simulink model "s_c_nbe_m32k"  (R2018a)
settings: Solver=VariableStepDiscrete  StartTime=0.0  StopTime=1000  RelTol=1e-3
undefined symbols (not defined in the file): fft_stages, n_taps, output_bits, pfb_coeff_gen_calc, xengbits
libraries: xbsIndex_r4 x23714, casper_library_misc x17, xps_library x4, casper_library_scopes x4, xbsReplacements_r4 x4
(part 125 of 171)

== system s_c_nbe_m32k/nb_pfb/pfb_fir_generic2/pfb_fir_taps/tap_delays ==
  addra : Inport
  dina : Inport  Port=2
  wea : Inport  Port=3
  addrb : Inport  Port=4
  dinb : Inport  Port=5
  web : Inport  Port=6
  A_bussify0 : Subsystem  mask(bus_create){inputNum=108}
      mask prompts: inputNum "Number of inputs:"
      mask init:
      | bus_create_init(gcb,...
      |     'inputNum', inputNum);
  B_bussify0 : Subsystem  mask(bus_create){inputNum=108}
      mask prompts: inputNum "Number of inputs:"
      mask init:
      | bus_create_init(gcb,...
      |     'inputNum', inputNum);
  alsbs_slice : xbsIndex_r4/Slice  nbits=15  boolean_output=off  mode=Lower Bit Location + Width  bit1=0  base1=LSB of Input  bit0=0  base0=LSB of Input  dbl_ovrd=off  block_type=slice
  blsbs_slice : xbsIndex_r4/Slice  nbits=15  boolean_output=off  mode=Lower Bit Location + Width  bit1=0  base1=LSB of Input  bit0=0  base0=LSB of Input  dbl_ovrd=off  block_type=slice
  bram0_{0..107} (108 alike) : xbsIndex_r4/Dual Port RAM  depth=32768  initVector=getfield(get_param(gcb, 'UserData'), 'initVector')  distributed_mem=Block RAM  init_a=0  init_b=0  rst_a=off  rst_b=off  en_a=off  en_b=off  latency=7  write_mode_A=Read Before Write  write_mode_B=Read Before Write  optimize=Speed  dbl_ovrd=off  block_type=dpram
  ddina0 : xbsIndex_r4/Delay  rst=off  infoeditControl=Selection of Reset will increase slice count due to use of real FFs and instead of SRLs  en=off  latency=0  reg_retiming=on  dbl_ovrd=off  block_type=delay
  ddinb0 : xbsIndex_r4/Delay  rst=off  infoeditControl=Selection of Reset will increase slice count due to use of real FFs and instead of SRLs  en=off  latency=4  reg_retiming=off  dbl_ovrd=off  block_type=delay
  debus_addra0 : Subsystem  mask(bus_expand){mode=divisions of equal size, outputNum=108, outputWidth=[15 15 15 15 15 15 15 15 15 15 15 15 15 15 15 15 15 15 15 15 15 15 15 15 15 15 15 15 15 15 15 15 15 15 15 15 15 15 15 15 15 15 15 15 15 15 15 15 15 15 15 15 15 15 15 15 15 15 15 15 15 15 15 15 15 15 15 15 15 15 15 15 15 15 15 15 15 15 15 15 15 15 15 15 15 15 15 15 15 15 15 15 15 15 15 15 15 15 15 15 15 15 15 15 15 15 15 15], outputBinaryPt=[0 0 0 0 0 0 0 0 0 0 0 0 0 0 0 0 0 0 0 0 0 0 0 0 0 0 0 0 0 0 0 0 0 0 0 0 0 0 0 0 0 0 0 0 0 0 0 0 0 0 0 0 0 0 0 0 0 0 0 0 0 0 0 0 0 0 0 0 0 0 0 0 0 0 0 0 0 0 0 0 0 0 0 0 0 0 0 0 0 0 0 0 0 0 0 0 0 0 0 0 0 0 0 0 0 0 0 0], outputArithmeticType=[0 0 0 0 0 0 0 0 0 0 0 0 0 0 0 0 0 0 0 0 0 0 0 0 0 0 0 0 0 0 0 0 0 0 0 0 0 0 0 0 0 0 0 0 0 0 0 0 0 0 0 0 0 0 0 0 0 0 0 0 0 0 0 0 0 0 0 0 0 0 0 0 0 0 0 0 0 0 0 0 0 0 0 0 0 0 0 0 0 0 0 0 0 0 0 0 0 0 0 0 0 0 0 0 0 0 0 0], show_format=on, outputToWorkspace=off, variablePrefix=, outputToModelAsWell=on}
      mask prompts: outputNum "Number of outputs:"; outputWidth "Output width:"; outputBinaryPt "Output binary point position:"; outputArithmeticType "Output arithmetic type (ufix=0, fix=1, bool=2):"; show_format "Print format string?"; outputToWorkspace "Output to workspace?"; variablePrefix "Variable name prefix:"; outputToModelAsWell "Output to model as well?"
      mask help:
      | Expands a 'bus' made using a bus_create or Xilinx
      | concat block.
      | The input will be divided into the specified number
      | of outputs with the specified arithmetic types.
      | Divisions are made from most significant bit.
      mask init: same as s_c_nbe_m32k/bus_expand1
      settings: AttributesFormatString=108 outputs: uf15.0,uf15.0,uf15.0,uf15.0,uf15.0,uf15.0,uf15.0,uf15.0,uf15.0,uf15.0,uf15.0,uf15.0,uf15.0,uf15.0,uf15.0,uf15.0,uf15.0,uf15.0,uf15.0,uf15.0,uf15.0,uf15.0,uf15.0,uf15.0,uf15.0,uf15.0,uf15.0,uf15.0,uf15.0,uf15.0,uf15.0,uf15.0,uf15.0,uf15.0,uf15.0,uf15.0,uf15.0,uf15.0,uf15.0,uf15.0,uf15.0,uf15.0,uf15.0,uf15.0,uf15.0,uf15.0,uf15.0,uf15.0,uf15.0,uf15.0,uf15.0,uf15.0,uf15.0,uf15.0,uf15.0,uf15.0,uf15.0,uf15.0,uf15.0,uf15.0,uf15.0,uf15.0,uf15.0,uf15.0,uf15.0,uf15.0,uf15.0,uf15.0,uf15.0,uf15.0,uf15.0,uf15.0,uf15.0,uf15.0,uf15.0,uf15.0,uf15.0,uf15.0,uf15.0,uf15.0,uf15.0,uf15.0,uf15.0,uf15.0,uf15.0,uf15.0,uf15.0,uf15.0,uf15.0,uf15.0,uf15.0,uf15.0,uf15.0,uf15.0,uf15.0,uf15.0,uf15.0,uf15.0,uf15.0,uf15.0,uf15.0,uf15.0,uf15.0,uf15.0,uf15.0,uf15.0,uf15.0,uf15.0,
      mask TypeOptions mode: divisions of equal size | divisions of arbitrary size
      mask Callback mode: bus_expand_callback();
      mask Callback outputWidth: bus_expand_callback();
      mask Callback outputToWorkspace: bus_expand_callback();
  debus_addrb0 : Subsystem  mask(bus_expand){mode=divisions of equal size, outputNum=108, outputWidth=[15 15 15 15 15 15 15 15 15 15 15 15 15 15 15 15 15 15 15 15 15 15 15 15 15 15 15 15 15 15 15 15 15 15 15 15 15 15 15 15 15 15 15 15 15 15 15 15 15 15 15 15 15 15 15 15 15 15 15 15 15 15 15 15 15 15 15 15 15 15 15 15 15 15 15 15 15 15 15 15 15 15 15 15 15 15 15 15 15 15 15 15 15 15 15 15 15 15 15 15 15 15 15 15 15 15 15 15], outputBinaryPt=[0 0 0 0 0 0 0 0 0 0 0 0 0 0 0 0 0 0 0 0 0 0 0 0 0 0 0 0 0 0 0 0 0 0 0 0 0 0 0 0 0 0 0 0 0 0 0 0 0 0 0 0 0 0 0 0 0 0 0 0 0 0 0 0 0 0 0 0 0 0 0 0 0 0 0 0 0 0 0 0 0 0 0 0 0 0 0 0 0 0 0 0 0 0 0 0 0 0 0 0 0 0 0 0 0 0 0 0], outputArithmeticType=[0 0 0 0 0 0 0 0 0 0 0 0 0 0 0 0 0 0 0 0 0 0 0 0 0 0 0 0 0 0 0 0 0 0 0 0 0 0 0 0 0 0 0 0 0 0 0 0 0 0 0 0 0 0 0 0 0 0 0 0 0 0 0 0 0 0 0 0 0 0 0 0 0 0 0 0 0 0 0 0 0 0 0 0 0 0 0 0 0 0 0 0 0 0 0 0 0 0 0 0 0 0 0 0 0 0 0 0], show_format=on, outputToWorkspace=off, variablePrefix=, outputToModelAsWell=on}
      mask prompts: outputNum "Number of outputs:"; outputWidth "Output width:"; outputBinaryPt "Output binary point position:"; outputArithmeticType "Output arithmetic type (ufix=0, fix=1, bool=2):"; show_format "Print format string?"; outputToWorkspace "Output to workspace?"; variablePrefix "Variable name prefix:"; outputToModelAsWell "Output to model as well?"
      mask help:
      | Expands a 'bus' made using a bus_create or Xilinx
      | concat block.
      | The input will be divided into the specified number
      | of outputs with the specified arithmetic types.
      | Divisions are made from most significant bit.
      mask init: same as s_c_nbe_m32k/bus_expand1
      settings: AttributesFormatString=108 outputs: uf15.0,uf15.0,uf15.0,uf15.0,uf15.0,uf15.0,uf15.0,uf15.0,uf15.0,uf15.0,uf15.0,uf15.0,uf15.0,uf15.0,uf15.0,uf15.0,uf15.0,uf15.0,uf15.0,uf15.0,uf15.0,uf15.0,uf15.0,uf15.0,uf15.0,uf15.0,uf15.0,uf15.0,uf15.0,uf15.0,uf15.0,uf15.0,uf15.0,uf15.0,uf15.0,uf15.0,uf15.0,uf15.0,uf15.0,uf15.0,uf15.0,uf15.0,uf15.0,uf15.0,uf15.0,uf15.0,uf15.0,uf15.0,uf15.0,uf15.0,uf15.0,uf15.0,uf15.0,uf15.0,uf15.0,uf15.0,uf15.0,uf15.0,uf15.0,uf15.0,uf15.0,uf15.0,uf15.0,uf15.0,uf15.0,uf15.0,uf15.0,uf15.0,uf15.0,uf15.0,uf15.0,uf15.0,uf15.0,uf15.0,uf15.0,uf15.0,uf15.0,uf15.0,uf15.0,uf15.0,uf15.0,uf15.0,uf15.0,uf15.0,uf15.0,uf15.0,uf15.0,uf15.0,uf15.0,uf15.0,uf15.0,uf15.0,uf15.0,uf15.0,uf15.0,uf15.0,uf15.0,uf15.0,uf15.0,uf15.0,uf15.0,uf15.0,uf15.0,uf15.0,uf15.0,uf15.0,uf15.0,uf15.0,
      mask TypeOptions mode: divisions of equal size | divisions of arbitrary size
      mask Callback mode: bus_expand_callback();
      mask Callback outputWidth: bus_expand_callback();
      mask Callback outputToWorkspace: bus_expand_callback();
  debus_dina0 : Subsystem  mask(bus_expand){mode=divisions of arbitrary size, outputNum=1, outputWidth=[1 1 1 1 1 1 1 1 1 1 1 1 1 1 1 1 1 1 1 1 1 1 1 1 1 1 1 1 1 1 1 1 1 1 1 1 1 1 1 1 1 1 1 1 1 1 1 1 1 1 1 1 1 1 1 1 1 1 1 1 1 1 1 1 1 1 1 1 1 1 1 1 1 1 1 1 1 1 1 1 1 1 1 1 1 1 1 1 1 1 1 1 1 1 1 1 1 1 1 1 1 1 1 1 1 1 1 1], outputBinaryPt=[0 0 0 0 0 0 0 0 0 0 0 0 0 0 0 0 0 0 0 0 0 0 0 0 0 0 0 0 0 0 0 0 0 0 0 0 0 0 0 0 0 0 0 0 0 0 0 0 0 0 0 0 0 0 0 0 0 0 0 0 0 0 0 0 0 0 0 0 0 0 0 0 0 0 0 0 0 0 0 0 0 0 0 0 0 0 0 0 0 0 0 0 0 0 0 0 0 0 0 0 0 0 0 0 0 0 0 0], outputArithmeticType=[0 0 0 0 0 0 0 0 0 0 0 0 0 0 0 0 0 0 0 0 0 0 0 0 0 0 0 0 0 0 0 0 0 0 0 0 0 0 0 0 0 0 0 0 0 0 0 0 0 0 0 0 0 0 0 0 0 0 0 0 0 0 0 0 0 0 0 0 0 0 0 0 0 0 0 0 0 0 0 0 0 0 0 0 0 0 0 0 0 0 0 0 0 0 0 0 0 0 0 0 0 0 0 0 0 0 0 0], show_format=on, outputToWorkspace=off, variablePrefix=, outputToModelAsWell=on}
      mask prompts: outputNum "Number of outputs:"; outputWidth "Output width [msb ... lsb]:"; outputBinaryPt "Output binary point position [msb ... lsb]:"; outputArithmeticType "Output arithmetic type (ufix=0, fix=1, bool=2) [msb ... lsb]:"; show_format "Print format string?"; outputToWorkspace "Output to workspace?"; variablePrefix "Variable name prefix:"; outputToModelAsWell "Output to model as well?"
      mask help:
      | Expands a 'bus' made using a bus_create or Xilinx
      | concat block.
      | The input will be divided into the specified number
      | of outputs with the specified arithmetic types.
      | Divisions are made from most significant bit.
      mask init: same as s_c_nbe_m32k/bus_expand1
      settings: AttributesFormatString=108 outputs: uf1.0,uf1.0,uf1.0,uf1.0,uf1.0,uf1.0,uf1.0,uf1.0,uf1.0,uf1.0,uf1.0,uf1.0,uf1.0,uf1.0,uf1.0,uf1.0,uf1.0,uf1.0,uf1.0,uf1.0,uf1.0,uf1.0,uf1.0,uf1.0,uf1.0,uf1.0,uf1.0,uf1.0,uf1.0,uf1.0,uf1.0,uf1.0,uf1.0,uf1.0,uf1.0,uf1.0,uf1.0,uf1.0,uf1.0,uf1.0,uf1.0,uf1.0,uf1.0,uf1.0,uf1.0,uf1.0,uf1.0,uf1.0,uf1.0,uf1.0,uf1.0,uf1.0,uf1.0,uf1.0,uf1.0,uf1.0,uf1.0,uf1.0,uf1.0,uf1.0,uf1.0,uf1.0,uf1.0,uf1.0,uf1.0,uf1.0,uf1.0,uf1.0,uf1.0,uf1.0,uf1.0,uf1.0,uf1.0,uf1.0,uf1.0,uf1.0,uf1.0,uf1.0,uf1.0,uf1.0,uf1.0,uf1.0,uf1.0,uf1.0,uf1.0,uf1.0,uf1.0,uf1.0,uf1.0,uf1.0,uf1.0,uf1.0,uf1.0,uf1.0,uf1.0,uf1.0,uf1.0,uf1.0,uf1.0,uf1.0,uf1.0,uf1.0,uf1.0,uf1.0,uf1.0,uf1.0,uf1.0,uf1.0,
      mask TypeOptions mode: divisions of equal size | divisions of arbitrary size
      mask Callback mode: bus_expand_callback();
      mask Callback outputWidth: bus_expand_callback();
      mask Callback outputToWorkspace: bus_expand_callback();
  debus_dinb0 : Subsystem  mask(bus_expand){mode=divisions of arbitrary size, outputNum=1, outputWidth=[1 1 1 1 1 1 1 1 1 1 1 1 1 1 1 1 1 1 1 1 1 1 1 1 1 1 1 1 1 1 1 1 1 1 1 1 1 1 1 1 1 1 1 1 1 1 1 1 1 1 1 1 1 1 1 1 1 1 1 1 1 1 1 1 1 1 1 1 1 1 1 1 1 1 1 1 1 1 1 1 1 1 1 1 1 1 1 1 1 1 1 1 1 1 1 1 1 1 1 1 1 1 1 1 1 1 1 1], outputBinaryPt=[0 0 0 0 0 0 0 0 0 0 0 0 0 0 0 0 0 0 0 0 0 0 0 0 0 0 0 0 0 0 0 0 0 0 0 0 0 0 0 0 0 0 0 0 0 0 0 0 0 0 0 0 0 0 0 0 0 0 0 0 0 0 0 0 0 0 0 0 0 0 0 0 0 0 0 0 0 0 0 0 0 0 0 0 0 0 0 0 0 0 0 0 0 0 0 0 0 0 0 0 0 0 0 0 0 0 0 0], outputArithmeticType=[0 0 0 0 0 0 0 0 0 0 0 0 0 0 0 0 0 0 0 0 0 0 0 0 0 0 0 0 0 0 0 0 0 0 0 0 0 0 0 0 0 0 0 0 0 0 0 0 0 0 0 0 0 0 0 0 0 0 0 0 0 0 0 0 0 0 0 0 0 0 0 0 0 0 0 0 0 0 0 0 0 0 0 0 0 0 0 0 0 0 0 0 0 0 0 0 0 0 0 0 0 0 0 0 0 0 0 0], show_format=on, outputToWorkspace=off, variablePrefix=, outputToModelAsWell=on}
      mask prompts: outputNum "Number of outputs:"; outputWidth "Output width [msb ... lsb]:"; outputBinaryPt "Output binary point position [msb ... lsb]:"; outputArithmeticType "Output arithmetic type (ufix=0, fix=1, bool=2) [msb ... lsb]:"; show_format "Print format string?"; outputToWorkspace "Output to workspace?"; variablePrefix "Variable name prefix:"; outputToModelAsWell "Output to model as well?"
      mask help:
      | Expands a 'bus' made using a bus_create or Xilinx
      | concat block.
      | The input will be divided into the specified number
      | of outputs with the specified arithmetic types.
      | Divisions are made from most significant bit.
      mask init: same as s_c_nbe_m32k/bus_expand1
      settings: AttributesFormatString=108 outputs: uf1.0,uf1.0,uf1.0,uf1.0,uf1.0,uf1.0,uf1.0,uf1.0,uf1.0,uf1.0,uf1.0,uf1.0,uf1.0,uf1.0,uf1.0,uf1.0,uf1.0,uf1.0,uf1.0,uf1.0,uf1.0,uf1.0,uf1.0,uf1.0,uf1.0,uf1.0,uf1.0,uf1.0,uf1.0,uf1.0,uf1.0,uf1.0,uf1.0,uf1.0,uf1.0,uf1.0,uf1.0,uf1.0,uf1.0,uf1.0,uf1.0,uf1.0,uf1.0,uf1.0,uf1.0,uf1.0,uf1.0,uf1.0,uf1.0,uf1.0,uf1.0,uf1.0,uf1.0,uf1.0,uf1.0,uf1.0,uf1.0,uf1.0,uf1.0,uf1.0,uf1.0,uf1.0,uf1.0,uf1.0,uf1.0,uf1.0,uf1.0,uf1.0,uf1.0,uf1.0,uf1.0,uf1.0,uf1.0,uf1.0,uf1.0,uf1.0,uf1.0,uf1.0,uf1.0,uf1.0,uf1.0,uf1.0,uf1.0,uf1.0,uf1.0,uf1.0,uf1.0,uf1.0,uf1.0,uf1.0,uf1.0,uf1.0,uf1.0,uf1.0,uf1.0,uf1.0,uf1.0,uf1.0,uf1.0,uf1.0,uf1.0,uf1.0,uf1.0,uf1.0,uf1.0,uf1.0,uf1.0,uf1.0,
      mask TypeOptions mode: divisions of equal size | divisions of arbitrary size
      mask Callback mode: bus_expand_callback();
      mask Callback outputWidth: bus_expand_callback();
      mask Callback outputToWorkspace: bus_expand_callback();
  debus_wea0 : Subsystem  mask(bus_expand){mode=divisions of equal size, outputNum=108, outputWidth=[1 1 1 1 1 1 1 1 1 1 1 1 1 1 1 1 1 1 1 1 1 1 1 1 1 1 1 1 1 1 1 1 1 1 1 1 1 1 1 1 1 1 1 1 1 1 1 1 1 1 1 1 1 1 1 1 1 1 1 1 1 1 1 1 1 1 1 1 1 1 1 1 1 1 1 1 1 1 1 1 1 1 1 1 1 1 1 1 1 1 1 1 1 1 1 1 1 1 1 1 1 1 1 1 1 1 1 1], outputBinaryPt=[0 0 0 0 0 0 0 0 0 0 0 0 0 0 0 0 0 0 0 0 0 0 0 0 0 0 0 0 0 0 0 0 0 0 0 0 0 0 0 0 0 0 0 0 0 0 0 0 0 0 0 0 0 0 0 0 0 0 0 0 0 0 0 0 0 0 0 0 0 0 0 0 0 0 0 0 0 0 0 0 0 0 0 0 0 0 0 0 0 0 0 0 0 0 0 0 0 0 0 0 0 0 0 0 0 0 0 0], outputArithmeticType=[2 2 2 2 2 2 2 2 2 2 2 2 2 2 2 2 2 2 2 2 2 2 2 2 2 2 2 2 2 2 2 2 2 2 2 2 2 2 2 2 2 2 2 2 2 2 2 2 2 2 2 2 2 2 2 2 2 2 2 2 2 2 2 2 2 2 2 2 2 2 2 2 2 2 2 2 2 2 2 2 2 2 2 2 2 2 2 2 2 2 2 2 2 2 2 2 2 2 2 2 2 2 2 2 2 2 2 2], show_format=on, outputToWorkspace=off, variablePrefix=, outputToModelAsWell=on}
      mask prompts: outputNum "Number of outputs:"; outputWidth "Output width:"; outputBinaryPt "Output binary point position:"; outputArithmeticType "Output arithmetic type (ufix=0, fix=1, bool=2):"; show_format "Print format string?"; outputToWorkspace "Output to workspace?"; variablePrefix "Variable name prefix:"; outputToModelAsWell "Output to model as well?"
      mask help:
      | Expands a 'bus' made using a bus_create or Xilinx
      | concat block.
      | The input will be divided into the specified number
      | of outputs with the specified arithmetic types.
      | Divisions are made from most significant bit.
      mask init: same as s_c_nbe_m32k/bus_expand1
      settings: AttributesFormatString=108 outputs: b,b,b,b,b,b,b,b,b,b,b,b,b,b,b,b,b,b,b,b,b,b,b,b,b,b,b,b,b,b,b,b,b,b,b,b,b,b,b,b,b,b,b,b,b,b,b,b,b,b,b,b,b,b,b,b,b,b,b,b,b,b,b,b,b,b,b,b,b,b,b,b,b,b,b,b,b,b,b,b,b,b,b,b,b,b,b,b,b,b,b,b,b,b,b,b,b,b,b,b,b,b,b,b,b,b,b,b,
      mask TypeOptions mode: divisions of equal size | divisions of arbitrary size
      mask Callback mode: bus_expand_callback();
      mask Callback outputWidth: bus_expand_callback();
      mask Callback outputToWorkspace: bus_expand_callback();
  debus_web0 : Subsystem  mask(bus_expand){mode=divisions of equal size, outputNum=108, outputWidth=[1 1 1 1 1 1 1 1 1 1 1 1 1 1 1 1 1 1 1 1 1 1 1 1 1 1 1 1 1 1 1 1 1 1 1 1 1 1 1 1 1 1 1 1 1 1 1 1 1 1 1 1 1 1 1 1 1 1 1 1 1 1 1 1 1 1 1 1 1 1 1 1 1 1 1 1 1 1 1 1 1 1 1 1 1 1 1 1 1 1 1 1 1 1 1 1 1 1 1 1 1 1 1 1 1 1 1 1], outputBinaryPt=[0 0 0 0 0 0 0 0 0 0 0 0 0 0 0 0 0 0 0 0 0 0 0 0 0 0 0 0 0 0 0 0 0 0 0 0 0 0 0 0 0 0 0 0 0 0 0 0 0 0 0 0 0 0 0 0 0 0 0 0 0 0 0 0 0 0 0 0 0 0 0 0 0 0 0 0 0 0 0 0 0 0 0 0 0 0 0 0 0 0 0 0 0 0 0 0 0 0 0 0 0 0 0 0 0 0 0 0], outputArithmeticType=[2 2 2 2 2 2 2 2 2 2 2 2 2 2 2 2 2 2 2 2 2 2 2 2 2 2 2 2 2 2 2 2 2 2 2 2 2 2 2 2 2 2 2 2 2 2 2 2 2 2 2 2 2 2 2 2 2 2 2 2 2 2 2 2 2 2 2 2 2 2 2 2 2 2 2 2 2 2 2 2 2 2 2 2 2 2 2 2 2 2 2 2 2 2 2 2 2 2 2 2 2 2 2 2 2 2 2 2], show_format=on, outputToWorkspace=off, variablePrefix=, outputToModelAsWell=on}
      mask prompts: outputNum "Number of outputs:"; outputWidth "Output width:"; outputBinaryPt "Output binary point position:"; outputArithmeticType "Output arithmetic type (ufix=0, fix=1, bool=2):"; show_format "Print format string?"; outputToWorkspace "Output to workspace?"; variablePrefix "Variable name prefix:"; outputToModelAsWell "Output to model as well?"
      mask help:
      | Expands a 'bus' made using a bus_create or Xilinx
      | concat block.
      | The input will be divided into the specified number
      | of outputs with the specified arithmetic types.
      | Divisions are made from most significant bit.
      mask init: same as s_c_nbe_m32k/bus_expand1
      settings: AttributesFormatString=108 outputs: b,b,b,b,b,b,b,b,b,b,b,b,b,b,b,b,b,b,b,b,b,b,b,b,b,b,b,b,b,b,b,b,b,b,b,b,b,b,b,b,b,b,b,b,b,b,b,b,b,b,b,b,b,b,b,b,b,b,b,b,b,b,b,b,b,b,b,b,b,b,b,b,b,b,b,b,b,b,b,b,b,b,b,b,b,b,b,b,b,b,b,b,b,b,b,b,b,b,b,b,b,b,b,b,b,b,b,b,
      mask TypeOptions mode: divisions of equal size | divisions of arbitrary size
      mask Callback mode: bus_expand_callback();
      mask Callback outputWidth: bus_expand_callback();
      mask Callback outputToWorkspace: bus_expand_callback();
  rep_addra0 : Subsystem  mask(bus_replicate){replication=108, csp_latency=4, misc=off, implementation=core}
      mask prompts: replication "replication factor"; csp_latency "latency"; misc "misc support"; implementation "delay implementation"
      mask help: Output bus formed by replicating input bus a number of times
      mask init:
      | bus_replicate_init(gcb, ...
      |     'replication', replication, ...
      |     'csp_latency', csp_latency, ...
      |     'implementation', implementation, ...
      |     'misc', misc);
      mask TypeOptions implementation: core | behavioral
  rep_addrb0 : Subsystem  mask(bus_replicate){replication=108, csp_latency=4, misc=off, implementation=core}
      mask prompts: replication "replication factor"; csp_latency "latency"; misc "misc support"; implementation "delay implementation"
      mask help: Output bus formed by replicating input bus a number of times
      mask init:
      | bus_replicate_init(gcb, ...
      |     'replication', replication, ...
      |     'csp_latency', csp_latency, ...
      |     'implementation', implementation, ...
      |     'misc', misc);
      mask TypeOptions implementation: core | behavioral
  rep_wea0 : Subsystem  mask(bus_replicate){replication=108, csp_latency=0, misc=off, implementation=behavioral}
      mask prompts: replication "replication factor"; csp_latency "latency"; misc "misc support"; implementation "delay implementation"
      mask help: Output bus formed by replicating input bus a number of times
      mask init:
      | bus_replicate_init(gcb, ...
      |     'replication', replication, ...
      |     'csp_latency', csp_latency, ...
      |     'implementation', implementation, ...
      |     'misc', misc);
      mask TypeOptions implementation: core | behavioral
  rep_web0 : Subsystem  mask(bus_replicate){replication=108, csp_latency=4, misc=off, implementation=core}
      mask prompts: replication "replication factor"; csp_latency "latency"; misc "misc support"; implementation "delay implementation"
      mask help: Output bus formed by replicating input bus a number of times
      mask init:
      | bus_replicate_init(gcb, ...
      |     'replication', replication, ...
      |     'csp_latency', csp_latency, ...
      |     'implementation', implementation, ...
      |     'misc', misc);
      mask TypeOptions implementation: core | behavioral
  A : Outport
  B : Outport  Port=2
  wires:
  B_bussify0/1(bus_out) -> B/1
  A_bussify0/1(bus_out) -> A/1
  bram0_107/2 -> B_bussify0/108(in108)
  bram0_107/1 -> A_bussify0/108(in108)
  bram0_106/2 -> B_bussify0/107(in107)
  bram0_106/1 -> A_bussify0/107(in107)
  bram0_105/2 -> B_bussify0/106(in106)
  bram0_105/1 -> A_bussify0/106(in106)
  bram0_104/2 -> B_bussify0/105(in105)
  bram0_104/1 -> A_bussify0/105(in105)
  bram0_103/2 -> B_bussify0/104(in104)
  bram0_103/1 -> A_bussify0/104(in104)
  bram0_102/2 -> B_bussify0/103(in103)
  bram0_102/1 -> A_bussify0/103(in103)
  bram0_101/2 -> B_bussify0/102(in102)
  bram0_101/1 -> A_bussify0/102(in102)
  bram0_100/2 -> B_bussify0/101(in101)
  bram0_100/1 -> A_bussify0/101(in101)
  bram0_99/2 -> B_bussify0/100(in100)
  bram0_99/1 -> A_bussify0/100(in100)
  bram0_98/2 -> B_bussify0/99(in99)
  bram0_98/1 -> A_bussify0/99(in99)
  bram0_97/2 -> B_bussify0/98(in98)
  bram0_97/1 -> A_bussify0/98(in98)
  bram0_96/2 -> B_bussify0/97(in97)
  bram0_96/1 -> A_bussify0/97(in97)
  bram0_95/2 -> B_bussify0/96(in96)
  bram0_95/1 -> A_bussify0/96(in96)
  bram0_94/2 -> B_bussify0/95(in95)
  bram0_94/1 -> A_bussify0/95(in95)
  bram0_93/2 -> B_bussify0/94(in94)
  bram0_93/1 -> A_bussify0/94(in94)
  bram0_92/2 -> B_bussify0/93(in93)
  bram0_92/1 -> A_bussify0/93(in93)
  bram0_91/2 -> B_bussify0/92(in92)
  bram0_91/1 -> A_bussify0/92(in92)
  bram0_90/2 -> B_bussify0/91(in91)
  bram0_90/1 -> A_bussify0/91(in91)
  bram0_89/2 -> B_bussify0/90(in90)
  bram0_89/1 -> A_bussify0/90(in90)
  bram0_88/2 -> B_bussify0/89(in89)
  bram0_88/1 -> A_bussify0/89(in89)
  bram0_87/2 -> B_bussify0/88(in88)
  bram0_87/1 -> A_bussify0/88(in88)
  bram0_86/2 -> B_bussify0/87(in87)
  bram0_86/1 -> A_bussify0/87(in87)
  bram0_85/2 -> B_bussify0/86(in86)
  bram0_85/1 -> A_bussify0/86(in86)
  bram0_84/2 -> B_bussify0/85(in85)
  bram0_84/1 -> A_bussify0/85(in85)
  bram0_83/2 -> B_bussify0/84(in84)
  bram0_83/1 -> A_bussify0/84(in84)
  bram0_82/2 -> B_bussify0/83(in83)
  bram0_82/1 -> A_bussify0/83(in83)
  bram0_81/2 -> B_bussify0/82(in82)
  bram0_81/1 -> A_bussify0/82(in82)
  bram0_80/2 -> B_bussify0/81(in81)
  bram0_80/1 -> A_bussify0/81(in81)
  bram0_79/2 -> B_bussify0/80(in80)
  bram0_79/1 -> A_bussify0/80(in80)
  bram0_78/2 -> B_bussify0/79(in79)
  bram0_78/1 -> A_bussify0/79(in79)
  bram0_77/2 -> B_bussify0/78(in78)
  bram0_77/1 -> A_bussify0/78(in78)
  bram0_76/2 -> B_bussify0/77(in77)
  bram0_76/1 -> A_bussify0/77(in77)
  bram0_75/2 -> B_bussify0/76(in76)
  bram0_75/1 -> A_bussify0/76(in76)
  bram0_74/2 -> B_bussify0/75(in75)
  bram0_74/1 -> A_bussify0/75(in75)
  bram0_73/2 -> B_bussify0/74(in74)
  bram0_73/1 -> A_bussify0/74(in74)
  bram0_72/2 -> B_bussify0/73(in73)
  bram0_72/1 -> A_bussify0/73(in73)
  bram0_71/2 -> B_bussify0/72(in72)
  bram0_71/1 -> A_bussify0/72(in72)
  bram0_70/2 -> B_bussify0/71(in71)
  bram0_70/1 -> A_bussify0/71(in71)
  bram0_69/2 -> B_bussify0/70(in70)
  bram0_69/1 -> A_bussify0/70(in70)
  bram0_68/2 -> B_bussify0/69(in69)
  bram0_68/1 -> A_bussify0/69(in69)
  bram0_67/2 -> B_bussify0/68(in68)
  bram0_67/1 -> A_bussify0/68(in68)
  bram0_66/2 -> B_bussify0/67(in67)
  bram0_66/1 -> A_bussify0/67(in67)
  bram0_65/2 -> B_bussify0/66(in66)
  bram0_65/1 -> A_bussify0/66(in66)
  bram0_64/2 -> B_bussify0/65(in65)
  bram0_64/1 -> A_bussify0/65(in65)
  bram0_63/2 -> B_bussify0/64(in64)
  bram0_63/1 -> A_bussify0/64(in64)
  bram0_62/2 -> B_bussify0/63(in63)
  bram0_62/1 -> A_bussify0/63(in63)
  bram0_61/2 -> B_bussify0/62(in62)
  bram0_61/1 -> A_bussify0/62(in62)
  bram0_60/2 -> B_bussify0/61(in61)
  bram0_60/1 -> A_bussify0/61(in61)
  bram0_59/2 -> B_bussify0/60(in60)
  bram0_59/1 -> A_bussify0/60(in60)
  bram0_58/2 -> B_bussify0/59(in59)
  bram0_58/1 -> A_bussify0/59(in59)
  bram0_57/2 -> B_bussify0/58(in58)
  bram0_57/1 -> A_bussify0/58(in58)
  bram0_56/2 -> B_bussify0/57(in57)
  bram0_56/1 -> A_bussify0/57(in57)
  bram0_55/2 -> B_bussify0/56(in56)
  bram0_55/1 -> A_bussify0/56(in56)
  bram0_54/2 -> B_bussify0/55(in55)
  bram0_54/1 -> A_bussify0/55(in55)
  bram0_53/2 -> B_bussify0/54(in54)
  bram0_53/1 -> A_bussify0/54(in54)
  bram0_52/2 -> B_bussify0/53(in53)
  bram0_52/1 -> A_bussify0/53(in53)
  bram0_51/2 -> B_bussify0/52(in52)
  bram0_51/1 -> A_bussify0/52(in52)
  bram0_50/2 -> B_bussify0/51(in51)
  bram0_50/1 -> A_bussify0/51(in51)
  bram0_49/2 -> B_bussify0/50(in50)
  bram0_49/1 -> A_bussify0/50(in50)
  bram0_48/2 -> B_bussify0/49(in49)
  bram0_48/1 -> A_bussify0/49(in49)
  bram0_47/2 -> B_bussify0/48(in48)
  bram0_47/1 -> A_bussify0/48(in48)
  bram0_46/2 -> B_bussify0/47(in47)
  bram0_46/1 -> A_bussify0/47(in47)
  bram0_45/2 -> B_bussify0/46(in46)
  bram0_45/1 -> A_bussify0/46(in46)
  bram0_44/2 -> B_bussify0/45(in45)
  bram0_44/1 -> A_bussify0/45(in45)
  bram0_43/2 -> B_bussify0/44(in44)
  bram0_43/1 -> A_bussify0/44(in44)
  bram0_42/2 -> B_bussify0/43(in43)
  bram0_42/1 -> A_bussify0/43(in43)
  bram0_41/2 -> B_bussify0/42(in42)
  bram0_41/1 -> A_bussify0/42(in42)
  bram0_40/2 -> B_bussify0/41(in41)
  bram0_40/1 -> A_bussify0/41(in41)
  bram0_39/2 -> B_bussify0/40(in40)
  bram0_39/1 -> A_bussify0/40(in40)
  bram0_38/2 -> B_bussify0/39(in39)
  bram0_38/1 -> A_bussify0/39(in39)
  bram0_37/2 -> B_bussify0/38(in38)
  bram0_37/1 -> A_bussify0/38(in38)
  bram0_36/2 -> B_bussify0/37(in37)
  bram0_36/1 -> A_bussify0/37(in37)
  bram0_35/2 -> B_bussify0/36(in36)
  bram0_35/1 -> A_bussify0/36(in36)
  bram0_34/2 -> B_bussify0/35(in35)
  bram0_34/1 -> A_bussify0/35(in35)
  bram0_33/2 -> B_bussify0/34(in34)
  bram0_33/1 -> A_bussify0/34(in34)
  bram0_32/2 -> B_bussify0/33(in33)
  bram0_32/1 -> A_bussify0/33(in33)
  bram0_31/2 -> B_bussify0/32(in32)
  bram0_31/1 -> A_bussify0/32(in32)
  bram0_30/2 -> B_bussify0/31(in31)
  bram0_30/1 -> A_bussify0/31(in31)
  bram0_29/2 -> B_bussify0/30(in30)
  bram0_29/1 -> A_bussify0/30(in30)
  bram0_28/2 -> B_bussify0/29(in29)
  bram0_28/1 -> A_bussify0/29(in29)
  bram0_27/2 -> B_bussify0/28(in28)
  bram0_27/1 -> A_bussify0/28(in28)
  bram0_26/2 -> B_bussify0/27(in27)
  bram0_26/1 -> A_bussify0/27(in27)
  bram0_25/2 -> B_bussify0/26(in26)
  bram0_25/1 -> A_bussify0/26(in26)
  bram0_24/2 -> B_bussify0/25(in25)
  bram0_24/1 -> A_bussify0/25(in25)
  bram0_23/2 -> B_bussify0/24(in24)
  bram0_23/1 -> A_bussify0/24(in24)
  bram0_22/2 -> B_bussify0/23(in23)
  bram0_22/1 -> A_bussify0/23(in23)
  bram0_21/2 -> B_bussify0/22(in22)
  bram0_21/1 -> A_bussify0/22(in22)
  bram0_20/2 -> B_bussify0/21(in21)
  bram0_20/1 -> A_bussify0/21(in21)
  bram0_19/2 -> B_bussify0/20(in20)
  bram0_19/1 -> A_bussify0/20(in20)
  bram0_18/2 -> B_bussify0/19(in19)
  bram0_18/1 -> A_bussify0/19(in19)
  bram0_17/2 -> B_bussify0/18(in18)
  bram0_17/1 -> A_bussify0/18(in18)
  bram0_16/2 -> B_bussify0/17(in17)
  bram0_16/1 -> A_bussify0/17(in17)
  bram0_15/2 -> B_bussify0/16(in16)
  bram0_15/1 -> A_bussify0/16(in16)
  bram0_14/2 -> B_bussify0/15(in15)
  bram0_14/1 -> A_bussify0/15(in15)
  bram0_13/2 -> B_bussify0/14(in14)
  bram0_13/1 -> A_bussify0/14(in14)
  bram0_12/2 -> B_bussify0/13(in13)
  bram0_12/1 -> A_bussify0/13(in13)
  bram0_11/2 -> B_bussify0/12(in12)
  bram0_11/1 -> A_bussify0/12(in12)
  bram0_10/2 -> B_bussify0/11(in11)
  bram0_10/1 -> A_bussify0/11(in11)
  bram0_9/2 -> B_bussify0/10(in10)
  bram0_9/1 -> A_bussify0/10(in10)
  bram0_8/2 -> B_bussify0/9(in9)
  bram0_8/1 -> A_bussify0/9(in9)
  bram0_7/2 -> B_bussify0/8(in8)
  bram0_7/1 -> A_bussify0/8(in8)
  bram0_6/2 -> B_bussify0/7(in7)
  bram0_6/1 -> A_bussify0/7(in7)
  bram0_5/2 -> B_bussify0/6(in6)
  bram0_5/1 -> A_bussify0/6(in6)
  bram0_4/2 -> B_bussify0/5(in5)
  bram0_4/1 -> A_bussify0/5(in5)
  bram0_3/2 -> B_bussify0/4(in4)
  bram0_3/1 -> A_bussify0/4(in4)
  bram0_2/2 -> B_bussify0/3(in3)
  bram0_2/1 -> A_bussify0/3(in3)
  bram0_1/2 -> B_bussify0/2(in2)
  bram0_1/1 -> A_bussify0/2(in2)
  bram0_0/2 -> B_bussify0/1(in1)
  bram0_0/1 -> A_bussify0/1(in1)
  debus_web0/108(lsb_out1) -> bram0_107/6
  debus_dinb0/108(lsb_out1) -> bram0_107/5
  debus_addrb0/108(lsb_out1) -> bram0_107/4
  debus_wea0/108(lsb_out1) -> bram0_107/3
  debus_dina0/108(lsb_out1) -> bram0_107/2
  debus_addra0/108(lsb_out1) -> bram0_107/1
  debus_web0/107(out2) -> bram0_106/6
  debus_dinb0/107(out2) -> bram0_106/5
  debus_addrb0/107(out2) -> bram0_106/4
  debus_wea0/107(out2) -> bram0_106/3
  debus_dina0/107(out2) -> bram0_106/2
  debus_addra0/107(out2) -> bram0_106/1
  debus_web0/106(out3) -> bram0_105/6
  debus_dinb0/106(out3) -> bram0_105/5
  debus_addrb0/106(out3) -> bram0_105/4
  debus_wea0/106(out3) -> bram0_105/3
  debus_dina0/106(out3) -> bram0_105/2
  debus_addra0/106(out3) -> bram0_105/1
  debus_web0/105(out4) -> bram0_104/6
  debus_dinb0/105(out4) -> bram0_104/5
  debus_addrb0/105(out4) -> bram0_104/4
  debus_wea0/105(out4) -> bram0_104/3
  debus_dina0/105(out4) -> bram0_104/2
  debus_addra0/105(out4) -> bram0_104/1
  debus_web0/104(out5) -> bram0_103/6
  debus_dinb0/104(out5) -> bram0_103/5
  debus_addrb0/104(out5) -> bram0_103/4
  debus_wea0/104(out5) -> bram0_103/3
  debus_dina0/104(out5) -> bram0_103/2
  debus_addra0/104(out5) -> bram0_103/1
  debus_web0/103(out6) -> bram0_102/6
  debus_dinb0/103(out6) -> bram0_102/5
  debus_addrb0/103(out6) -> bram0_102/4
  debus_wea0/103(out6) -> bram0_102/3
  debus_dina0/103(out6) -> bram0_102/2
  debus_addra0/103(out6) -> bram0_102/1
  debus_web0/102(out7) -> bram0_101/6
  debus_dinb0/102(out7) -> bram0_101/5
  debus_addrb0/102(out7) -> bram0_101/4
  debus_wea0/102(out7) -> bram0_101/3
  debus_dina0/102(out7) -> bram0_101/2
  debus_addra0/102(out7) -> bram0_101/1
  debus_web0/101(out8) -> bram0_100/6
  debus_dinb0/101(out8) -> bram0_100/5
  debus_addrb0/101(out8) -> bram0_100/4
  debus_wea0/101(out8) -> bram0_100/3
  debus_dina0/101(out8) -> bram0_100/2
  debus_addra0/101(out8) -> bram0_100/1
  debus_web0/100(out9) -> bram0_99/6
  debus_dinb0/100(out9) -> bram0_99/5
  debus_addrb0/100(out9) -> bram0_99/4
  debus_wea0/100(out9) -> bram0_99/3
  debus_dina0/100(out9) -> bram0_99/2
  debus_addra0/100(out9) -> bram0_99/1
  debus_web0/99(out10) -> bram0_98/6
  debus_dinb0/99(out10) -> bram0_98/5
  debus_addrb0/99(out10) -> bram0_98/4
  debus_wea0/99(out10) -> bram0_98/3
  debus_dina0/99(out10) -> bram0_98/2
  debus_addra0/99(out10) -> bram0_98/1
  debus_web0/98(out11) -> bram0_97/6
  debus_dinb0/98(out11) -> bram0_97/5
  debus_addrb0/98(out11) -> bram0_97/4
  debus_wea0/98(out11) -> bram0_97/3
  debus_dina0/98(out11) -> bram0_97/2
  debus_addra0/98(out11) -> bram0_97/1
  debus_web0/97(out12) -> bram0_96/6
  debus_dinb0/97(out12) -> bram0_96/5
  debus_addrb0/97(out12) -> bram0_96/4
  debus_wea0/97(out12) -> bram0_96/3
  debus_dina0/97(out12) -> bram0_96/2
  debus_addra0/97(out12) -> bram0_96/1
  debus_web0/96(out13) -> bram0_95/6
  debus_dinb0/96(out13) -> bram0_95/5
  debus_addrb0/96(out13) -> bram0_95/4
  debus_wea0/96(out13) -> bram0_95/3
  debus_dina0/96(out13) -> bram0_95/2
  debus_addra0/96(out13) -> bram0_95/1
  debus_web0/95(out14) -> bram0_94/6
  debus_dinb0/95(out14) -> bram0_94/5
  debus_addrb0/95(out14) -> bram0_94/4
  debus_wea0/95(out14) -> bram0_94/3
  debus_dina0/95(out14) -> bram0_94/2
  debus_addra0/95(out14) -> bram0_94/1
  debus_web0/94(out15) -> bram0_93/6
  debus_dinb0/94(out15) -> bram0_93/5
  debus_addrb0/94(out15) -> bram0_93/4
  debus_wea0/94(out15) -> bram0_93/3
  debus_dina0/94(out15) -> bram0_93/2
  debus_addra0/94(out15) -> bram0_93/1
  debus_web0/93(out16) -> bram0_92/6
  debus_dinb0/93(out16) -> bram0_92/5
  debus_addrb0/93(out16) -> bram0_92/4
  debus_wea0/93(out16) -> bram0_92/3
  debus_dina0/93(out16) -> bram0_92/2
  debus_addra0/93(out16) -> bram0_92/1
  debus_web0/92(out17) -> bram0_91/6
  debus_dinb0/92(out17) -> bram0_91/5
  debus_addrb0/92(out17) -> bram0_91/4
  debus_wea0/92(out17) -> bram0_91/3
  debus_dina0/92(out17) -> bram0_91/2
  debus_addra0/92(out17) -> bram0_91/1
  debus_web0/91(out18) -> bram0_90/6
  debus_dinb0/91(out18) -> bram0_90/5
  debus_addrb0/91(out18) -> bram0_90/4
  debus_wea0/91(out18) -> bram0_90/3
  debus_dina0/91(out18) -> bram0_90/2
  debus_addra0/91(out18) -> bram0_90/1
  debus_web0/90(out19) -> bram0_89/6
  debus_dinb0/90(out19) -> bram0_89/5
  debus_addrb0/90(out19) -> bram0_89/4
  debus_wea0/90(out19) -> bram0_89/3
  debus_dina0/90(out19) -> bram0_89/2
  debus_addra0/90(out19) -> bram0_89/1
  debus_web0/89(out20) -> bram0_88/6
  debus_dinb0/89(out20) -> bram0_88/5
  debus_addrb0/89(out20) -> bram0_88/4
  debus_wea0/89(out20) -> bram0_88/3
  debus_dina0/89(out20) -> bram0_88/2
  debus_addra0/89(out20) -> bram0_88/1
  debus_web0/88(out21) -> bram0_87/6
  debus_dinb0/88(out21) -> bram0_87/5
  debus_addrb0/88(out21) -> bram0_87/4
  debus_wea0/88(out21) -> bram0_87/3
  debus_dina0/88(out21) -> bram0_87/2
  debus_addra0/88(out21) -> bram0_87/1
  debus_web0/87(out22) -> bram0_86/6
  debus_dinb0/87(out22) -> bram0_86/5
  debus_addrb0/87(out22) -> bram0_86/4
  debus_wea0/87(out22) -> bram0_86/3
  debus_dina0/87(out22) -> bram0_86/2
  debus_addra0/87(out22) -> bram0_86/1
  debus_web0/86(out23) -> bram0_85/6
  debus_dinb0/86(out23) -> bram0_85/5
  debus_addrb0/86(out23) -> bram0_85/4
  debus_wea0/86(out23) -> bram0_85/3
  debus_dina0/86(out23) -> bram0_85/2
  debus_addra0/86(out23) -> bram0_85/1
  debus_web0/85(out24) -> bram0_84/6
  debus_dinb0/85(out24) -> bram0_84/5
  debus_addrb0/85(out24) -> bram0_84/4
  debus_wea0/85(out24) -> bram0_84/3
  debus_dina0/85(out24) -> bram0_84/2
  debus_addra0/85(out24) -> bram0_84/1
  debus_web0/84(out25) -> bram0_83/6
  debus_dinb0/84(out25) -> bram0_83/5
  debus_addrb0/84(out25) -> bram0_83/4
  debus_wea0/84(out25) -> bram0_83/3
  debus_dina0/84(out25) -> bram0_83/2
  debus_addra0/84(out25) -> bram0_83/1
  debus_web0/83(out26) -> bram0_82/6
  debus_dinb0/83(out26) -> bram0_82/5
  debus_addrb0/83(out26) -> bram0_82/4
  debus_wea0/83(out26) -> bram0_82/3
  debus_dina0/83(out26) -> bram0_82/2
  debus_addra0/83(out26) -> bram0_82/1
  debus_web0/82(out27) -> bram0_81/6
  debus_dinb0/82(out27) -> bram0_81/5
  debus_addrb0/82(out27) -> bram0_81/4
  debus_wea0/82(out27) -> bram0_81/3
  debus_dina0/82(out27) -> bram0_81/2
  debus_addra0/82(out27) -> bram0_81/1
  debus_web0/81(out28) -> bram0_80/6
  debus_dinb0/81(out28) -> bram0_80/5
  debus_addrb0/81(out28) -> bram0_80/4
  debus_wea0/81(out28) -> bram0_80/3
  debus_dina0/81(out28) -> bram0_80/2
  debus_addra0/81(out28) -> bram0_80/1
  debus_web0/80(out29) -> bram0_79/6
  debus_dinb0/80(out29) -> bram0_79/5
  debus_addrb0/80(out29) -> bram0_79/4
  debus_wea0/80(out29) -> bram0_79/3
  debus_dina0/80(out29) -> bram0_79/2
  debus_addra0/80(out29) -> bram0_79/1
  debus_web0/79(out30) -> bram0_78/6
  debus_dinb0/79(out30) -> bram0_78/5
  debus_addrb0/79(out30) -> bram0_78/4
  debus_wea0/79(out30) -> bram0_78/3
  debus_dina0/79(out30) -> bram0_78/2
  debus_addra0/79(out30) -> bram0_78/1
  debus_web0/78(out31) -> bram0_77/6
  debus_dinb0/78(out31) -> bram0_77/5
  debus_addrb0/78(out31) -> bram0_77/4
  debus_wea0/78(out31) -> bram0_77/3
  debus_dina0/78(out31) -> bram0_77/2
  debus_addra0/78(out31) -> bram0_77/1
  debus_web0/77(out32) -> bram0_76/6
  debus_dinb0/77(out32) -> bram0_76/5
  debus_addrb0/77(out32) -> bram0_76/4
  debus_wea0/77(out32) -> bram0_76/3
  debus_dina0/77(out32) -> bram0_76/2
  debus_addra0/77(out32) -> bram0_76/1
  debus_web0/76(out33) -> bram0_75/6
  debus_dinb0/76(out33) -> bram0_75/5
  debus_addrb0/76(out33) -> bram0_75/4
  debus_wea0/76(out33) -> bram0_75/3
  debus_dina0/76(out33) -> bram0_75/2
  debus_addra0/76(out33) -> bram0_75/1
  debus_web0/75(out34) -> bram0_74/6
  debus_dinb0/75(out34) -> bram0_74/5
  debus_addrb0/75(out34) -> bram0_74/4
  debus_wea0/75(out34) -> bram0_74/3
  debus_dina0/75(out34) -> bram0_74/2
  debus_addra0/75(out34) -> bram0_74/1
  debus_web0/74(out35) -> bram0_73/6
  debus_dinb0/74(out35) -> bram0_73/5
  debus_addrb0/74(out35) -> bram0_73/4
  debus_wea0/74(out35) -> bram0_73/3
  debus_dina0/74(out35) -> bram0_73/2
  debus_addra0/74(out35) -> bram0_73/1
  debus_web0/73(out36) -> bram0_72/6
  debus_dinb0/73(out36) -> bram0_72/5
  debus_addrb0/73(out36) -> bram0_72/4
  debus_wea0/73(out36) -> bram0_72/3
  debus_dina0/73(out36) -> bram0_72/2
  debus_addra0/73(out36) -> bram0_72/1
  debus_web0/72(out37) -> bram0_71/6
  debus_dinb0/72(out37) -> bram0_71/5
  debus_addrb0/72(out37) -> bram0_71/4
  debus_wea0/72(out37) -> bram0_71/3
  debus_dina0/72(out37) -> bram0_71/2
  debus_addra0/72(out37) -> bram0_71/1
  debus_web0/71(out38) -> bram0_70/6
  debus_dinb0/71(out38) -> bram0_70/5
  debus_addrb0/71(out38) -> bram0_70/4
  debus_wea0/71(out38) -> bram0_70/3
  debus_dina0/71(out38) -> bram0_70/2
  debus_addra0/71(out38) -> bram0_70/1
  debus_web0/70(out39) -> bram0_69/6
  debus_dinb0/70(out39) -> bram0_69/5
  debus_addrb0/70(out39) -> bram0_69/4
  debus_wea0/70(out39) -> bram0_69/3
  debus_dina0/70(out39) -> bram0_69/2
  debus_addra0/70(out39) -> bram0_69/1
  debus_web0/69(out40) -> bram0_68/6
  debus_dinb0/69(out40) -> bram0_68/5
  debus_addrb0/69(out40) -> bram0_68/4
  debus_wea0/69(out40) -> bram0_68/3
  debus_dina0/69(out40) -> bram0_68/2
  debus_addra0/69(out40) -> bram0_68/1
  debus_web0/68(out41) -> bram0_67/6
  debus_dinb0/68(out41) -> bram0_67/5
  debus_addrb0/68(out41) -> bram0_67/4
  debus_wea0/68(out41) -> bram0_67/3
  debus_dina0/68(out41) -> bram0_67/2
  debus_addra0/68(out41) -> bram0_67/1
  debus_web0/67(out42) -> bram0_66/6
  debus_dinb0/67(out42) -> bram0_66/5
  debus_addrb0/67(out42) -> bram0_66/4
  debus_wea0/67(out42) -> bram0_66/3
  debus_dina0/67(out42) -> bram0_66/2
  debus_addra0/67(out42) -> bram0_66/1
  debus_web0/66(out43) -> bram0_65/6
  debus_dinb0/66(out43) -> bram0_65/5
  debus_addrb0/66(out43) -> bram0_65/4
  debus_wea0/66(out43) -> bram0_65/3
  debus_dina0/66(out43) -> bram0_65/2
  debus_addra0/66(out43) -> bram0_65/1
  debus_web0/65(out44) -> bram0_64/6
  debus_dinb0/65(out44) -> bram0_64/5
  debus_addrb0/65(out44) -> bram0_64/4
  debus_wea0/65(out44) -> bram0_64/3
  debus_dina0/65(out44) -> bram0_64/2
  debus_addra0/65(out44) -> bram0_64/1
  debus_web0/64(out45) -> bram0_63/6
  debus_dinb0/64(out45) -> bram0_63/5
  debus_addrb0/64(out45) -> bram0_63/4
  debus_wea0/64(out45) -> bram0_63/3
  debus_dina0/64(out45) -> bram0_63/2
  debus_addra0/64(out45) -> bram0_63/1
  debus_web0/63(out46) -> bram0_62/6
  debus_dinb0/63(out46) -> bram0_62/5
  debus_addrb0/63(out46) -> bram0_62/4
  debus_wea0/63(out46) -> bram0_62/3
  debus_dina0/63(out46) -> bram0_62/2
  debus_addra0/63(out46) -> bram0_62/1
  debus_web0/62(out47) -> bram0_61/6
  debus_dinb0/62(out47) -> bram0_61/5
  debus_addrb0/62(out47) -> bram0_61/4
  debus_wea0/62(out47) -> bram0_61/3
  debus_dina0/62(out47) -> bram0_61/2
  debus_addra0/62(out47) -> bram0_61/1
  debus_web0/61(out48) -> bram0_60/6
  debus_dinb0/61(out48) -> bram0_60/5
  debus_addrb0/61(out48) -> bram0_60/4
  debus_wea0/61(out48) -> bram0_60/3
  debus_dina0/61(out48) -> bram0_60/2
  debus_addra0/61(out48) -> bram0_60/1
  debus_web0/60(out49) -> bram0_59/6
  debus_dinb0/60(out49) -> bram0_59/5
  debus_addrb0/60(out49) -> bram0_59/4
  debus_wea0/60(out49) -> bram0_59/3
  debus_dina0/60(out49) -> bram0_59/2
  debus_addra0/60(out49) -> bram0_59/1
  debus_web0/59(out50) -> bram0_58/6
  debus_dinb0/59(out50) -> bram0_58/5
  debus_addrb0/59(out50) -> bram0_58/4
  debus_wea0/59(out50) -> bram0_58/3
  debus_dina0/59(out50) -> bram0_58/2
  debus_addra0/59(out50) -> bram0_58/1
  debus_web0/58(out51) -> bram0_57/6
  debus_dinb0/58(out51) -> bram0_57/5
  debus_addrb0/58(out51) -> bram0_57/4
  debus_wea0/58(out51) -> bram0_57/3
  debus_dina0/58(out51) -> bram0_57/2
  debus_addra0/58(out51) -> bram0_57/1
  debus_web0/57(out52) -> bram0_56/6
  debus_dinb0/57(out52) -> bram0_56/5
  debus_addrb0/57(out52) -> bram0_56/4
  debus_wea0/57(out52) -> bram0_56/3
  debus_dina0/57(out52) -> bram0_56/2
  debus_addra0/57(out52) -> bram0_56/1
  debus_web0/56(out53) -> bram0_55/6
  debus_dinb0/56(out53) -> bram0_55/5
  debus_addrb0/56(out53) -> bram0_55/4
  debus_wea0/56(out53) -> bram0_55/3
  debus_dina0/56(out53) -> bram0_55/2
  debus_addra0/56(out53) -> bram0_55/1
  debus_web0/55(out54) -> bram0_54/6
  debus_dinb0/55(out54) -> bram0_54/5
  debus_addrb0/55(out54) -> bram0_54/4
  debus_wea0/55(out54) -> bram0_54/3
  debus_dina0/55(out54) -> bram0_54/2
  debus_addra0/55(out54) -> bram0_54/1
  debus_web0/54(out55) -> bram0_53/6
  debus_dinb0/54(out55) -> bram0_53/5
  debus_addrb0/54(out55) -> bram0_53/4
  debus_wea0/54(out55) -> bram0_53/3
  debus_dina0/54(out55) -> bram0_53/2
  debus_addra0/54(out55) -> bram0_53/1
  debus_web0/53(out56) -> bram0_52/6
  debus_dinb0/53(out56) -> bram0_52/5
  debus_addrb0/53(out56) -> bram0_52/4
  debus_wea0/53(out56) -> bram0_52/3
  debus_dina0/53(out56) -> bram0_52/2
  debus_addra0/53(out56) -> bram0_52/1
  debus_web0/52(out57) -> bram0_51/6
  debus_dinb0/52(out57) -> bram0_51/5
  debus_addrb0/52(out57) -> bram0_51/4
  debus_wea0/52(out57) -> bram0_51/3
  debus_dina0/52(out57) -> bram0_51/2
  debus_addra0/52(out57) -> bram0_51/1
  debus_web0/51(out58) -> bram0_50/6
  debus_dinb0/51(out58) -> bram0_50/5
  debus_addrb0/51(out58) -> bram0_50/4
  debus_wea0/51(out58) -> bram0_50/3
  debus_dina0/51(out58) -> bram0_50/2
  debus_addra0/51(out58) -> bram0_50/1
  debus_web0/50(out59) -> bram0_49/6
  debus_dinb0/50(out59) -> bram0_49/5
  debus_addrb0/50(out59) -> bram0_49/4
  debus_wea0/50(out59) -> bram0_49/3
  debus_dina0/50(out59) -> bram0_49/2
  debus_addra0/50(out59) -> bram0_49/1
  debus_web0/49(out60) -> bram0_48/6
  debus_dinb0/49(out60) -> bram0_48/5
  debus_addrb0/49(out60) -> bram0_48/4
  debus_wea0/49(out60) -> bram0_48/3
  debus_dina0/49(out60) -> bram0_48/2
  debus_addra0/49(out60) -> bram0_48/1
  debus_web0/48(out61) -> bram0_47/6
  debus_dinb0/48(out61) -> bram0_47/5
  debus_addrb0/48(out61) -> bram0_47/4
  debus_wea0/48(out61) -> bram0_47/3
  debus_dina0/48(out61) -> bram0_47/2
  debus_addra0/48(out61) -> bram0_47/1
  debus_web0/47(out62) -> bram0_46/6
  debus_dinb0/47(out62) -> bram0_46/5
  debus_addrb0/47(out62) -> bram0_46/4
  debus_wea0/47(out62) -> bram0_46/3
  debus_dina0/47(out62) -> bram0_46/2
  debus_addra0/47(out62) -> bram0_46/1
  debus_web0/46(out63) -> bram0_45/6
  debus_dinb0/46(out63) -> bram0_45/5
  debus_addrb0/46(out63) -> bram0_45/4
  debus_wea0/46(out63) -> bram0_45/3
  debus_dina0/46(out63) -> bram0_45/2
  debus_addra0/46(out63) -> bram0_45/1
  debus_web0/45(out64) -> bram0_44/6
  debus_dinb0/45(out64) -> bram0_44/5
  debus_addrb0/45(out64) -> bram0_44/4
  debus_wea0/45(out64) -> bram0_44/3
  debus_dina0/45(out64) -> bram0_44/2
  debus_addra0/45(out64) -> bram0_44/1
  debus_web0/44(out65) -> bram0_43/6
  debus_dinb0/44(out65) -> bram0_43/5
  debus_addrb0/44(out65) -> bram0_43/4
  debus_wea0/44(out65) -> bram0_43/3
  debus_dina0/44(out65) -> bram0_43/2
  debus_addra0/44(out65) -> bram0_43/1
  debus_web0/43(out66) -> bram0_42/6
  debus_dinb0/43(out66) -> bram0_42/5
  debus_addrb0/43(out66) -> bram0_42/4
  debus_wea0/43(out66) -> bram0_42/3
  debus_dina0/43(out66) -> bram0_42/2
  debus_addra0/43(out66) -> bram0_42/1
  debus_web0/42(out67) -> bram0_41/6
  debus_dinb0/42(out67) -> bram0_41/5
  debus_addrb0/42(out67) -> bram0_41/4
  debus_wea0/42(out67) -> bram0_41/3
  debus_dina0/42(out67) -> bram0_41/2
  debus_addra0/42(out67) -> bram0_41/1
  debus_web0/41(out68) -> bram0_40/6
  debus_dinb0/41(out68) -> bram0_40/5
  debus_addrb0/41(out68) -> bram0_40/4
  debus_wea0/41(out68) -> bram0_40/3
  debus_dina0/41(out68) -> bram0_40/2
  debus_addra0/41(out68) -> bram0_40/1
  debus_web0/40(out69) -> bram0_39/6
  debus_dinb0/40(out69) -> bram0_39/5
  debus_addrb0/40(out69) -> bram0_39/4
  debus_wea0/40(out69) -> bram0_39/3
  debus_dina0/40(out69) -> bram0_39/2
  debus_addra0/40(out69) -> bram0_39/1
  debus_web0/39(out70) -> bram0_38/6
  debus_dinb0/39(out70) -> bram0_38/5
  debus_addrb0/39(out70) -> bram0_38/4
  debus_wea0/39(out70) -> bram0_38/3
  debus_dina0/39(out70) -> bram0_38/2
  debus_addra0/39(out70) -> bram0_38/1
  debus_web0/38(out71) -> bram0_37/6
  debus_dinb0/38(out71) -> bram0_37/5
  debus_addrb0/38(out71) -> bram0_37/4
  debus_wea0/38(out71) -> bram0_37/3
  debus_dina0/38(out71) -> bram0_37/2
  debus_addra0/38(out71) -> bram0_37/1
  debus_web0/37(out72) -> bram0_36/6
  debus_dinb0/37(out72) -> bram0_36/5
  debus_addrb0/37(out72) -> bram0_36/4
  debus_wea0/37(out72) -> bram0_36/3
  debus_dina0/37(out72) -> bram0_36/2
  debus_addra0/37(out72) -> bram0_36/1
  debus_web0/36(out73) -> bram0_35/6
  debus_dinb0/36(out73) -> bram0_35/5
  debus_addrb0/36(out73) -> bram0_35/4
  debus_wea0/36(out73) -> bram0_35/3
  debus_dina0/36(out73) -> bram0_35/2
  debus_addra0/36(out73) -> bram0_35/1
  debus_web0/35(out74) -> bram0_34/6
  debus_dinb0/35(out74) -> bram0_34/5
  debus_addrb0/35(out74) -> bram0_34/4
  debus_wea0/35(out74) -> bram0_34/3
  debus_dina0/35(out74) -> bram0_34/2
  debus_addra0/35(out74) -> bram0_34/1
  debus_web0/34(out75) -> bram0_33/6
  debus_dinb0/34(out75) -> bram0_33/5
  debus_addrb0/34(out75) -> bram0_33/4
  debus_wea0/34(out75) -> bram0_33/3
  debus_dina0/34(out75) -> bram0_33/2
  debus_addra0/34(out75) -> bram0_33/1
  debus_web0/33(out76) -> bram0_32/6
  debus_dinb0/33(out76) -> bram0_32/5
  debus_addrb0/33(out76) -> bram0_32/4
  debus_wea0/33(out76) -> bram0_32/3
  debus_dina0/33(out76) -> bram0_32/2
  debus_addra0/33(out76) -> bram0_32/1
  debus_web0/32(out77) -> bram0_31/6
  debus_dinb0/32(out77) -> bram0_31/5
  debus_addrb0/32(out77) -> bram0_31/4
  debus_wea0/32(out77) -> bram0_31/3
  debus_dina0/32(out77) -> bram0_31/2
  debus_addra0/32(out77) -> bram0_31/1
  debus_web0/31(out78) -> bram0_30/6
  debus_dinb0/31(out78) -> bram0_30/5
  debus_addrb0/31(out78) -> bram0_30/4
  debus_wea0/31(out78) -> bram0_30/3
  debus_dina0/31(out78) -> bram0_30/2
  debus_addra0/31(out78) -> bram0_30/1
  debus_web0/30(out79) -> bram0_29/6
  debus_dinb0/30(out79) -> bram0_29/5
  debus_addrb0/30(out79) -> bram0_29/4
  debus_wea0/30(out79) -> bram0_29/3
  debus_dina0/30(out79) -> bram0_29/2
  debus_addra0/30(out79) -> bram0_29/1
  debus_web0/29(out80) -> bram0_28/6
  debus_dinb0/29(out80) -> bram0_28/5
  debus_addrb0/29(out80) -> bram0_28/4
  debus_wea0/29(out80) -> bram0_28/3
  debus_dina0/29(out80) -> bram0_28/2
  debus_addra0/29(out80) -> bram0_28/1
  debus_web0/28(out81) -> bram0_27/6
  debus_dinb0/28(out81) -> bram0_27/5
  debus_addrb0/28(out81) -> bram0_27/4
  debus_wea0/28(out81) -> bram0_27/3
  debus_dina0/28(out81) -> bram0_27/2
  debus_addra0/28(out81) -> bram0_27/1
  debus_web0/27(out82) -> bram0_26/6
  debus_dinb0/27(out82) -> bram0_26/5
  debus_addrb0/27(out82) -> bram0_26/4
  debus_wea0/27(out82) -> bram0_26/3
  debus_dina0/27(out82) -> bram0_26/2
  debus_addra0/27(out82) -> bram0_26/1
  debus_web0/26(out83) -> bram0_25/6
  debus_dinb0/26(out83) -> bram0_25/5
  debus_addrb0/26(out83) -> bram0_25/4
  debus_wea0/26(out83) -> bram0_25/3
  debus_dina0/26(out83) -> bram0_25/2
  debus_addra0/26(out83) -> bram0_25/1
  debus_web0/25(out84) -> bram0_24/6
  debus_dinb0/25(out84) -> bram0_24/5
  debus_addrb0/25(out84) -> bram0_24/4
  debus_wea0/25(out84) -> bram0_24/3
  debus_dina0/25(out84) -> bram0_24/2
  debus_addra0/25(out84) -> bram0_24/1
  debus_web0/24(out85) -> bram0_23/6
  debus_dinb0/24(out85) -> bram0_23/5
  debus_addrb0/24(out85) -> bram0_23/4
  debus_wea0/24(out85) -> bram0_23/3
  debus_dina0/24(out85) -> bram0_23/2
  debus_addra0/24(out85) -> bram0_23/1
  debus_web0/23(out86) -> bram0_22/6
  debus_dinb0/23(out86) -> bram0_22/5
  debus_addrb0/23(out86) -> bram0_22/4
  debus_wea0/23(out86) -> bram0_22/3
  debus_dina0/23(out86) -> bram0_22/2
  debus_addra0/23(out86) -> bram0_22/1
  debus_web0/22(out87) -> bram0_21/6
  debus_dinb0/22(out87) -> bram0_21/5
  debus_addrb0/22(out87) -> bram0_21/4
  debus_wea0/22(out87) -> bram0_21/3
  debus_dina0/22(out87) -> bram0_21/2
  debus_addra0/22(out87) -> bram0_21/1
  debus_web0/21(out88) -> bram0_20/6
  debus_dinb0/21(out88) -> bram0_20/5
  debus_addrb0/21(out88) -> bram0_20/4
  debus_wea0/21(out88) -> bram0_20/3
  debus_dina0/21(out88) -> bram0_20/2
  debus_addra0/21(out88) -> bram0_20/1
  debus_web0/20(out89) -> bram0_19/6
  debus_dinb0/20(out89) -> bram0_19/5
  debus_addrb0/20(out89) -> bram0_19/4
  debus_wea0/20(out89) -> bram0_19/3
  debus_dina0/20(out89) -> bram0_19/2
  debus_addra0/20(out89) -> bram0_19/1
  debus_web0/19(out90) -> bram0_18/6
  debus_dinb0/19(out90) -> bram0_18/5
  debus_addrb0/19(out90) -> bram0_18/4
  debus_wea0/19(out90) -> bram0_18/3
  debus_dina0/19(out90) -> bram0_18/2
  debus_addra0/19(out90) -> bram0_18/1
  debus_web0/18(out91) -> bram0_17/6
  debus_dinb0/18(out91) -> bram0_17/5
  debus_addrb0/18(out91) -> bram0_17/4
  debus_wea0/18(out91) -> bram0_17/3
  debus_dina0/18(out91) -> bram0_17/2
  debus_addra0/18(out91) -> bram0_17/1
  debus_web0/17(out92) -> bram0_16/6
  debus_dinb0/17(out92) -> bram0_16/5
  debus_addrb0/17(out92) -> bram0_16/4
  debus_wea0/17(out92) -> bram0_16/3
  debus_dina0/17(out92) -> bram0_16/2
  debus_addra0/17(out92) -> bram0_16/1
  debus_web0/16(out93) -> bram0_15/6
  debus_dinb0/16(out93) -> bram0_15/5
  debus_addrb0/16(out93) -> bram0_15/4
  debus_wea0/16(out93) -> bram0_15/3
  debus_dina0/16(out93) -> bram0_15/2
  debus_addra0/16(out93) -> bram0_15/1
  debus_web0/15(out94) -> bram0_14/6
  debus_dinb0/15(out94) -> bram0_14/5
  debus_addrb0/15(out94) -> bram0_14/4
  debus_wea0/15(out94) -> bram0_14/3
  debus_dina0/15(out94) -> bram0_14/2
  debus_addra0/15(out94) -> bram0_14/1
  debus_web0/14(out95) -> bram0_13/6
  debus_dinb0/14(out95) -> bram0_13/5
  debus_addrb0/14(out95) -> bram0_13/4
  debus_wea0/14(out95) -> bram0_13/3
  debus_dina0/14(out95) -> bram0_13/2
  debus_addra0/14(out95) -> bram0_13/1
  debus_web0/13(out96) -> bram0_12/6
  debus_dinb0/13(out96) -> bram0_12/5
  debus_addrb0/13(out96) -> bram0_12/4
  debus_wea0/13(out96) -> bram0_12/3
  debus_dina0/13(out96) -> bram0_12/2
  debus_addra0/13(out96) -> bram0_12/1
  debus_web0/12(out97) -> bram0_11/6
  debus_dinb0/12(out97) -> bram0_11/5
  debus_addrb0/12(out97) -> bram0_11/4
  debus_wea0/12(out97) -> bram0_11/3
  debus_dina0/12(out97) -> bram0_11/2
  debus_addra0/12(out97) -> bram0_11/1
  debus_web0/11(out98) -> bram0_10/6
  debus_dinb0/11(out98) -> bram0_10/5
  debus_addrb0/11(out98) -> bram0_10/4
  debus_wea0/11(out98) -> bram0_10/3
  debus_dina0/11(out98) -> bram0_10/2
  debus_addra0/11(out98) -> bram0_10/1
  debus_web0/10(out99) -> bram0_9/6
  debus_dinb0/10(out99) -> bram0_9/5
  debus_addrb0/10(out99) -> bram0_9/4
  debus_wea0/10(out99) -> bram0_9/3
  debus_dina0/10(out99) -> bram0_9/2
  debus_addra0/10(out99) -> bram0_9/1
  debus_web0/9(out100) -> bram0_8/6
  debus_dinb0/9(out100) -> bram0_8/5
  debus_addrb0/9(out100) -> bram0_8/4
  debus_wea0/9(out100) -> bram0_8/3
  debus_dina0/9(out100) -> bram0_8/2
  debus_addra0/9(out100) -> bram0_8/1
  debus_web0/8(out101) -> bram0_7/6
  debus_dinb0/8(out101) -> bram0_7/5
  debus_addrb0/8(out101) -> bram0_7/4
  debus_wea0/8(out101) -> bram0_7/3
  debus_dina0/8(out101) -> bram0_7/2
  debus_addra0/8(out101) -> bram0_7/1
  debus_web0/7(out102) -> bram0_6/6
  debus_dinb0/7(out102) -> bram0_6/5
  debus_addrb0/7(out102) -> bram0_6/4
  debus_wea0/7(out102) -> bram0_6/3
  debus_dina0/7(out102) -> bram0_6/2
  debus_addra0/7(out102) -> bram0_6/1
  debus_web0/6(out103) -> bram0_5/6
  debus_dinb0/6(out103) -> bram0_5/5
  debus_addrb0/6(out103) -> bram0_5/4
  debus_wea0/6(out103) -> bram0_5/3
  debus_dina0/6(out103) -> bram0_5/2
  debus_addra0/6(out103) -> bram0_5/1
  debus_web0/5(out104) -> bram0_4/6
  debus_dinb0/5(out104) -> bram0_4/5
  debus_addrb0/5(out104) -> bram0_4/4
  debus_wea0/5(out104) -> bram0_4/3
  debus_dina0/5(out104) -> bram0_4/2
  debus_addra0/5(out104) -> bram0_4/1
  debus_web0/4(out105) -> bram0_3/6
  debus_dinb0/4(out105) -> bram0_3/5
  debus_addrb0/4(out105) -> bram0_3/4
  debus_wea0/4(out105) -> bram0_3/3
  debus_dina0/4(out105) -> bram0_3/2
  debus_addra0/4(out105) -> bram0_3/1
  debus_web0/3(out106) -> bram0_2/6
  debus_dinb0/3(out106) -> bram0_2/5
  debus_addrb0/3(out106) -> bram0_2/4
  debus_wea0/3(out106) -> bram0_2/3
  debus_dina0/3(out106) -> bram0_2/2
  debus_addra0/3(out106) -> bram0_2/1
  debus_web0/2(out107) -> bram0_1/6
  debus_dinb0/2(out107) -> bram0_1/5
  debus_addrb0/2(out107) -> bram0_1/4
  debus_wea0/2(out107) -> bram0_1/3
  debus_dina0/2(out107) -> bram0_1/2
  debus_addra0/2(out107) -> bram0_1/1
  debus_web0/1(msb_out108) -> bram0_0/6
  debus_dinb0/1(msb_out108) -> bram0_0/5
  debus_addrb0/1(msb_out108) -> bram0_0/4
  debus_wea0/1(msb_out108) -> bram0_0/3
  debus_dina0/1(msb_out108) -> bram0_0/2
  debus_addra0/1(msb_out108) -> bram0_0/1
  rep_web0/1(out) -> debus_web0/1(bus_in)
  ddinb0/1 -> debus_dinb0/1(bus_in)
  rep_wea0/1(out) -> debus_wea0/1(bus_in)
  ddina0/1 -> debus_dina0/1(bus_in)
  rep_addra0/1(out) -> debus_addra0/1(bus_in)
  rep_addrb0/1(out) -> debus_addrb0/1(bus_in)
  web/1 -> rep_web0/1(in)
  dinb/1 -> ddinb0/1
  wea/1 -> rep_wea0/1(in)
  dina/1 -> ddina0/1
  alsbs_slice/1 -> rep_addra0/1(in)
  blsbs_slice/1 -> rep_addrb0/1(in)
  addra/1 -> alsbs_slice/1
  addrb/1 -> blsbs_slice/1
